simulink model "KUKA_coupled_Dynamics"  (R2023a)
settings: Solver=ode4  StartTime=0.0  StopTime=10  FixedStep=0.01  RelTol=1e-3  EnableMultiTasking=on
InitFcn:
  | % ************** Initiate forces
  | % f0=[0;0;0;0;0;0];
  | % f0=[0;0;0;0;0;0;0];
  | %f_0=[0;0;0];
  | %f_m=[0;0];
  | %f_e=[0;0;0;0;0;0];
  | %iota0=eye(6);
  | % ************** Initiate states
  | %q_m=[2;1];
  | %q_dot_m=[0;1];
  | %P=[0;0;0];
  | %V_I0=[0;0;0];
  | % ************** Load main
  | %run(Main.m)
StopFcn:
  | %format long
  | %table(out.qddot.data(:,1)',out.qddot_ref.data(1,:))
values from neighbouring files (symbols this model uses):
  diag_M = diagonalize(M_frak0, M_frak)    [Create_Robot.m]    (also in Main.m; Main__iiwa7.m; diagonalize.m = zeros(6*(n+1),6*(n+1)); test_C_Main.m)
  f_0 = [0;0;0]    [Create_Robot.m]    (also in Main.m; Main__iiwa7.m = [0;0;0;0;0;0]; test_C_Main.m)
  f_m = [0;0]    [Create_Robot.m]    (also in Main.m; Main__iiwa7.m; test_C_Main.m)
  I0 = eye(3)*416.667    [Create_Robot.m]    (also in Main.m; Main__iiwa7.m = eye(3)*1.66667; test_C_Main.m)
  iota0 = [1 0 0; 0 1 0;zeros(3,3);0 0 1]    [Create_Robot.m]    (also in Main.m = [1 0 0 0 0 0; 0 1 0 0 0 0; 0 0 0 0 0 1]'; Main__iiwa7.m = eye(6,6); test_C_Main.m)
  m0 = 100    [Create_Robot.m]    (also in Main.m; Main__iiwa7.m = 10; test_C_Main.m)
  P = [0;0;0]    [Create_Robot.m]    (also in Main.m = M0*V_I0+M0m*q_dot_m; Main__iiwa7.m = M0*V_I0+M0m*q_dot_m; test_C_Main.m)
  q_dot_m = [0;0]    [Create_Robot.m]    (also in Main.m; Main__iiwa7.m; test_C_Main.m)
  q_m = [0;0]    [Create_Robot.m]    (also in Main.m = [0.2;0.4]; Main__iiwa7.m = [0.2;0.4]; test_C_Main.m = [1;0])
  X = [0 -x(3) x(2) ; x(3) 0 -x(1) ; -x(2) x(1) 0 ]    [skewsym.m]
  Xi_m_matrix = zeros(6*n,n)    [Create_Robot.m]    (also in Main.m; Main__iiwa7.m; test_C_Main.m)
undefined symbols (not defined in the file or in its folder): Xi_m, Y, Z
libraries: sm_lib x80, nesl_utility x36
(part 3 of 3)

== system KUKA_coupled_Dynamics/Space Manipulator1/joint//link6/iiwa_link_6 ==
  Inertia : sm_lib/Body Elements/Inertia  InertiaType=Custom  Mass=2.3466  MassUnits=kg  CenterOfMass=[0, 0, 0]  CenterOfMassUnits=m  MomentsOfInertia=[0.006509, 0.006259, 0.004527]  MomentsOfInertiaUnits=kg*m^2  ProductsOfInertia=[0.00031891, 0, 0]  ProductsOfInertiaUnits=kg*m^2  GraphicType=None  MarkerShape=Inertia  MarkerSize=20  GraphicVisPropType=SimpleVisualProperties  GraphicDiffuseColor=[0.5 0.5 0.5]  GraphicSpecularColor=[0.5 0.5 0.5 1.0]  GraphicAmbientColor=[0.15 0.15 0.15 1.0]  GraphicEmissiveColor=[0.0 0.0 0.0 1.0]  GraphicShininess=75  GraphicOpacity=1.0
  InertiaOriginTransform : sm_lib/Frames and Transforms/Rigid Transform  TranslationMethod=Cartesian  TranslationStandardOffset=0  TranslationStandardOffsetUnits=m  TranslationStandardAxis=+Z  TranslationCartesianOffset=[0, 0.0005999999999999999, 0.0004]  TranslationCartesianOffsetUnits=m  TranslationROffset=0  TranslationROffsetUnits=m  TranslationZOffset=0  TranslationZOffsetUnits=m  TranslationThetaOffset=0  TranslationThetaOffsetUnits=deg  RotationMethod=RotationSequence  RotationAngleUnits=deg  RotationStandardAxis=+Z  RotationAngle=0.0  RotationArbitraryAxis=[0 0 1]  FollAlignAxisA=+X  BaseAlignAxisA=+Y  FollAlignAxisB=+Y  BaseAlignAxisB=+Z  RotationSequenceAxes=BaseAxes  RotationSequence=XYZ  RotationSequenceAngles=[0, 0, 0]  RotationSequenceAnglesUnits=rad  RotationMatrix=[1 0 0; 0 1 0; 0 0 1]  Quaternion=[1 0 0 0]
  ReferenceFrame : sm_lib/Frames and Transforms/Reference Frame
  Visual : sm_lib/Body Elements/File Solid  ExtGeomFileName=iiwa_description/meshes/iiwa7/visual/link_6.stl  UnitType=Custom  ExtGeomFileUnits=m  StepReaderType=HEX  ExportConvexHullGeometry=off  InertiaType=Custom  Mass=0  MassUnits=kg  CenterOfMass=[0, 0, 0]  CenterOfMassUnits=m  MomentsOfInertia=[0, 0, 0]  MomentsOfInertiaUnits=kg*m^2  ProductsOfInertia=[0, 0, 0]  ProductsOfInertiaUnits=kg*m^2  BasedOnType=DensityFromFile  Density=1000  DensityUnits=kg/m^3  DoExposeReferenceFrame=on  SerializedFrames=<Frames/>  GraphicType=FromGeometry  MarkerShape=Sphere  MarkerSize=10  GraphicVisPropType=SimpleVisualProperties  GraphicDiffuseColor=[1, 0.423529411765, 0.0392156862745]  GraphicSpecularColor=[0.5 0.5 0.5 1.0]  GraphicAmbientColor=[0.15 0.15 0.15 1.0]  GraphicEmissiveColor=[0.0 0.0 0.0 1.0]  GraphicShininess=75  GraphicOpacity=1
  VisualOriginTransform : sm_lib/Frames and Transforms/Rigid Transform  TranslationMethod=Cartesian  TranslationStandardOffset=0  TranslationStandardOffsetUnits=m  TranslationStandardAxis=+Z  TranslationCartesianOffset=[0, 0, 0]  TranslationCartesianOffsetUnits=m  TranslationROffset=0  TranslationROffsetUnits=m  TranslationZOffset=0  TranslationZOffsetUnits=m  TranslationThetaOffset=0  TranslationThetaOffsetUnits=deg  RotationMethod=RotationSequence  RotationAngleUnits=deg  RotationStandardAxis=+Z  RotationAngle=0.0  RotationArbitraryAxis=[0 0 1]  FollAlignAxisA=+X  BaseAlignAxisA=+Y  FollAlignAxisB=+Y  BaseAlignAxisB=+Z  RotationSequenceAxes=BaseAxes  RotationSequence=XYZ  RotationSequenceAngles=[0, 0, 0]  RotationSequenceAnglesUnits=rad  RotationMatrix=[1 0 0; 0 1 0; 0 0 1]  Quaternion=[1 0 0 0]
  iiwa_joint_6_AxisInvTransform : sm_lib/Frames and Transforms/Rigid Transform  TranslationMethod=Cartesian  TranslationStandardOffset=0  TranslationStandardOffsetUnits=m  TranslationStandardAxis=+Z  TranslationCartesianOffset=[0, 0, 0]  TranslationCartesianOffsetUnits=m  TranslationROffset=0  TranslationROffsetUnits=m  TranslationZOffset=0  TranslationZOffsetUnits=m  TranslationThetaOffset=0  TranslationThetaOffsetUnits=deg  RotationMethod=ArbitraryAxis  RotationAngleUnits=rad  RotationStandardAxis=+Z  RotationAngle=0  RotationArbitraryAxis=[1, 0, 0]  FollAlignAxisA=+X  BaseAlignAxisA=+Y  FollAlignAxisB=+Y  BaseAlignAxisB=+Z  RotationSequenceAxes=FollowerAxes  RotationSequence=XYX  RotationSequenceAngles=[0 0 0]  RotationSequenceAnglesUnits=deg  RotationMatrix=[1 0 0; 0 1 0; 0 0 1]  Quaternion=[1 0 0 0]
  iiwa_joint_7_AxisTransform : sm_lib/Frames and Transforms/Rigid Transform  TranslationMethod=Cartesian  TranslationStandardOffset=0  TranslationStandardOffsetUnits=m  TranslationStandardAxis=+Z  TranslationCartesianOffset=[0, 0, 0]  TranslationCartesianOffsetUnits=m  TranslationROffset=0  TranslationROffsetUnits=m  TranslationZOffset=0  TranslationZOffsetUnits=m  TranslationThetaOffset=0  TranslationThetaOffsetUnits=deg  RotationMethod=ArbitraryAxis  RotationAngleUnits=rad  RotationStandardAxis=+Z  RotationAngle=0  RotationArbitraryAxis=[1, 0, 0]  FollAlignAxisA=+X  BaseAlignAxisA=+Y  FollAlignAxisB=+Y  BaseAlignAxisB=+Z  RotationSequenceAxes=FollowerAxes  RotationSequence=XYX  RotationSequenceAngles=[0 0 0]  RotationSequenceAnglesUnits=deg  RotationMatrix=[1 0 0; 0 1 0; 0 0 1]  Quaternion=[1 0 0 0]
  iiwa_joint_7_OriginTransform : sm_lib/Frames and Transforms/Rigid Transform  TranslationMethod=Cartesian  TranslationStandardOffset=0  TranslationStandardOffsetUnits=m  TranslationStandardAxis=+Z  TranslationCartesianOffset=[0, 0.081, 0.0607]  TranslationCartesianOffsetUnits=m  TranslationROffset=0  TranslationROffsetUnits=m  TranslationZOffset=0  TranslationZOffsetUnits=m  TranslationThetaOffset=0  TranslationThetaOffsetUnits=deg  RotationMethod=RotationSequence  RotationAngleUnits=deg  RotationStandardAxis=+Z  RotationAngle=0.0  RotationArbitraryAxis=[0 0 1]  FollAlignAxisA=+X  BaseAlignAxisA=+Y  FollAlignAxisB=+Y  BaseAlignAxisB=+Z  RotationSequenceAxes=BaseAxes  RotationSequence=XYZ  RotationSequenceAngles=[-1.57079632679, 3.14159265359, 0]  RotationSequenceAnglesUnits=rad  RotationMatrix=[1 0 0; 0 1 0; 0 0 1]  Quaternion=[1 0 0 0]
  F : PMIOPort  Side=Left
  F1 : PMIOPort  Port=2  Side=Right
  connections:
  Inertia/RConn1 -- InertiaOriginTransform/RConn1
  InertiaOriginTransform/LConn1 -- ReferenceFrame/RConn1 -- VisualOriginTransform/LConn1 -- iiwa_joint_6_AxisInvTransform/LConn1 -- iiwa_joint_7_OriginTransform/LConn1
  Visual/RConn1 -- VisualOriginTransform/RConn1
  iiwa_joint_6_AxisInvTransform/RConn1 -- F/RConn1
  iiwa_joint_7_AxisTransform/RConn1 -- F1/RConn1
  iiwa_joint_7_AxisTransform/LConn1 -- iiwa_joint_7_OriginTransform/RConn1

== system KUKA_coupled_Dynamics/Space Manipulator1/joint//link7/iiwa_link_7 ==
  Inertia : sm_lib/Body Elements/Inertia  InertiaType=Custom  Mass=3.129  MassUnits=kg  CenterOfMass=[0, 0, 0]  CenterOfMassUnits=m  MomentsOfInertia=[0.01464, 0.01465, 0.002872]  MomentsOfInertiaUnits=kg*m^2  ProductsOfInertia=[0, 0, 0.0005912]  ProductsOfInertiaUnits=kg*m^2  GraphicType=None  MarkerShape=Inertia  MarkerSize=20  GraphicVisPropType=SimpleVisualProperties  GraphicDiffuseColor=[0.5 0.5 0.5]  GraphicSpecularColor=[0.5 0.5 0.5 1.0]  GraphicAmbientColor=[0.15 0.15 0.15 1.0]  GraphicEmissiveColor=[0.0 0.0 0.0 1.0]  GraphicShininess=75  GraphicOpacity=1.0
  InertiaOriginTransform : sm_lib/Frames and Transforms/Rigid Transform  TranslationMethod=Cartesian  TranslationStandardOffset=0  TranslationStandardOffsetUnits=m  TranslationStandardAxis=+Z  TranslationCartesianOffset=[0, 0, 0.02]  TranslationCartesianOffsetUnits=m  TranslationROffset=0  TranslationROffsetUnits=m  TranslationZOffset=0  TranslationZOffsetUnits=m  TranslationThetaOffset=0  TranslationThetaOffsetUnits=deg  RotationMethod=RotationSequence  RotationAngleUnits=deg  RotationStandardAxis=+Z  RotationAngle=0.0  RotationArbitraryAxis=[0 0 1]  FollAlignAxisA=+X  BaseAlignAxisA=+Y  FollAlignAxisB=+Y  BaseAlignAxisB=+Z  RotationSequenceAxes=BaseAxes  RotationSequence=XYZ  RotationSequenceAngles=[0, 0, 0]  RotationSequenceAnglesUnits=rad  RotationMatrix=[1 0 0; 0 1 0; 0 0 1]  Quaternion=[1 0 0 0]
  ReferenceFrame : sm_lib/Frames and Transforms/Reference Frame
  Visual : sm_lib/Body Elements/File Solid  ExtGeomFileName=iiwa_description/meshes/iiwa7/visual/link_7.stl  UnitType=Custom  ExtGeomFileUnits=m  StepReaderType=HEX  ExportConvexHullGeometry=off  InertiaType=Custom  Mass=0  MassUnits=kg  CenterOfMass=[0, 0, 0]  CenterOfMassUnits=m  MomentsOfInertia=[0, 0, 0]  MomentsOfInertiaUnits=kg*m^2  ProductsOfInertia=[0, 0, 0]  ProductsOfInertiaUnits=kg*m^2  BasedOnType=DensityFromFile  Density=1000  DensityUnits=kg/m^3  DoExposeReferenceFrame=on  SerializedFrames=<Frames/>  GraphicType=FromGeometry  MarkerShape=Sphere  MarkerSize=10  GraphicVisPropType=SimpleVisualProperties  GraphicDiffuseColor=[0.4, 0.4, 0.4]  GraphicSpecularColor=[0.5 0.5 0.5 1.0]  GraphicAmbientColor=[0.15 0.15 0.15 1.0]  GraphicEmissiveColor=[0.0 0.0 0.0 1.0]  GraphicShininess=75  GraphicOpacity=1
  VisualOriginTransform : sm_lib/Frames and Transforms/Rigid Transform  TranslationMethod=Cartesian  TranslationStandardOffset=0  TranslationStandardOffsetUnits=m  TranslationStandardAxis=+Z  TranslationCartesianOffset=[0, 0, -0.0005]  TranslationCartesianOffsetUnits=m  TranslationROffset=0  TranslationROffsetUnits=m  TranslationZOffset=0  TranslationZOffsetUnits=m  TranslationThetaOffset=0  TranslationThetaOffsetUnits=deg  RotationMethod=RotationSequence  RotationAngleUnits=deg  RotationStandardAxis=+Z  RotationAngle=0.0  RotationArbitraryAxis=[0 0 1]  FollAlignAxisA=+X  BaseAlignAxisA=+Y  FollAlignAxisB=+Y  BaseAlignAxisB=+Z  RotationSequenceAxes=BaseAxes  RotationSequence=XYZ  RotationSequenceAngles=[0, 0, 0]  RotationSequenceAnglesUnits=rad  RotationMatrix=[1 0 0; 0 1 0; 0 0 1]  Quaternion=[1 0 0 0]
  iiwa_joint_7_AxisInvTransform : sm_lib/Frames and Transforms/Rigid Transform  TranslationMethod=Cartesian  TranslationStandardOffset=0  TranslationStandardOffsetUnits=m  TranslationStandardAxis=+Z  TranslationCartesianOffset=[0, 0, 0]  TranslationCartesianOffsetUnits=m  TranslationROffset=0  TranslationROffsetUnits=m  TranslationZOffset=0  TranslationZOffsetUnits=m  TranslationThetaOffset=0  TranslationThetaOffsetUnits=deg  RotationMethod=ArbitraryAxis  RotationAngleUnits=rad  RotationStandardAxis=+Z  RotationAngle=0  RotationArbitraryAxis=[1, 0, 0]  FollAlignAxisA=+X  BaseAlignAxisA=+Y  FollAlignAxisB=+Y  BaseAlignAxisB=+Z  RotationSequenceAxes=FollowerAxes  RotationSequence=XYX  RotationSequenceAngles=[0 0 0]  RotationSequenceAnglesUnits=deg  RotationMatrix=[1 0 0; 0 1 0; 0 0 1]  Quaternion=[1 0 0 0]
  iiwa_joint_ee_OriginTransform : sm_lib/Frames and Transforms/Rigid Transform  TranslationMethod=Cartesian  TranslationStandardOffset=0  TranslationStandardOffsetUnits=m  TranslationStandardAxis=+Z  TranslationCartesianOffset=[0, 0, 0.045]  TranslationCartesianOffsetUnits=m  TranslationROffset=0  TranslationROffsetUnits=m  TranslationZOffset=0  TranslationZOffsetUnits=m  TranslationThetaOffset=0  TranslationThetaOffsetUnits=deg  RotationMethod=RotationSequence  RotationAngleUnits=deg  RotationStandardAxis=+Z  RotationAngle=0.0  RotationArbitraryAxis=[0 0 1]  FollAlignAxisA=+X  BaseAlignAxisA=+Y  FollAlignAxisB=+Y  BaseAlignAxisB=+Z  RotationSequenceAxes=BaseAxes  RotationSequence=XYZ  RotationSequenceAngles=[0, -1.57079632679, 0]  RotationSequenceAnglesUnits=rad  RotationMatrix=[1 0 0; 0 1 0; 0 0 1]  Quaternion=[1 0 0 0]
  iiwa_joint_ee_kuka_OriginTransform : sm_lib/Frames and Transforms/Rigid Transform  TranslationMethod=Cartesian  TranslationStandardOffset=0  TranslationStandardOffsetUnits=m  TranslationStandardAxis=+Z  TranslationCartesianOffset=[0, 0, 0.045]  TranslationCartesianOffsetUnits=m  TranslationROffset=0  TranslationROffsetUnits=m  TranslationZOffset=0  TranslationZOffsetUnits=m  TranslationThetaOffset=0  TranslationThetaOffsetUnits=deg  RotationMethod=RotationSequence  RotationAngleUnits=deg  RotationStandardAxis=+Z  RotationAngle=0.0  RotationArbitraryAxis=[0 0 1]  FollAlignAxisA=+X  BaseAlignAxisA=+Y  FollAlignAxisB=+Y  BaseAlignAxisB=+Z  RotationSequenceAxes=BaseAxes  RotationSequence=XYZ  RotationSequenceAngles=[3.14159265359, 3.14159265359, 3.14159265359]  RotationSequenceAnglesUnits=rad  RotationMatrix=[1 0 0; 0 1 0; 0 0 1]  Quaternion=[1 0 0 0]
  F : PMIOPort  Side=Left
  F2 : PMIOPort  Port=2  Side=Right
  F1 : PMIOPort  Port=3  Side=Right
  connections:
  Inertia/RConn1 -- InertiaOriginTransform/RConn1
  InertiaOriginTransform/LConn1 -- iiwa_joint_ee_OriginTransform/LConn1 -- iiwa_joint_ee_kuka_OriginTransform/LConn1 -- iiwa_joint_7_AxisInvTransform/LConn1 -- VisualOriginTransform/LConn1 -- ReferenceFrame/RConn1
  Visual/RConn1 -- VisualOriginTransform/RConn1
  iiwa_joint_7_AxisInvTransform/RConn1 -- F/RConn1
  iiwa_joint_ee_OriginTransform/RConn1 -- F1/RConn1
  iiwa_joint_ee_kuka_OriginTransform/RConn1 -- F2/RConn1

== system KUKA_coupled_Dynamics/old model1/Inverse Dynamics/Euler Poincare ==
  P : Inport
  V : Inport  Port=2
  f_0 : Inport  Port=3
  Add : Sum  Inputs=+-
  Constant : Constant  Value=iota0
  MATLAB Function : MATLAB Function  TreatAsAtomicUnit=on
  Matrix Multiply : Product  Multiplication=Matrix(*)
  To Workspace : ToWorkspace  VariableName=simout  SaveFormat=Timeseries  SampleTime=-1
  Transpose : Math  Operator=transpose
  P_dot : Outport
  wires:
  P/1 -> Matrix Multiply/2
  MATLAB Function/1(adj_low) -> Transpose/1
  V/1 -> MATLAB Function/1(V)
  Transpose/1 -> To Workspace/1, Matrix Multiply/1
  Matrix Multiply/1 -> Add/1
  f_0/1 -> Add/2
  Add/1 -> P_dot/1
  Constant/1 -> MATLAB Function/2(iota0)

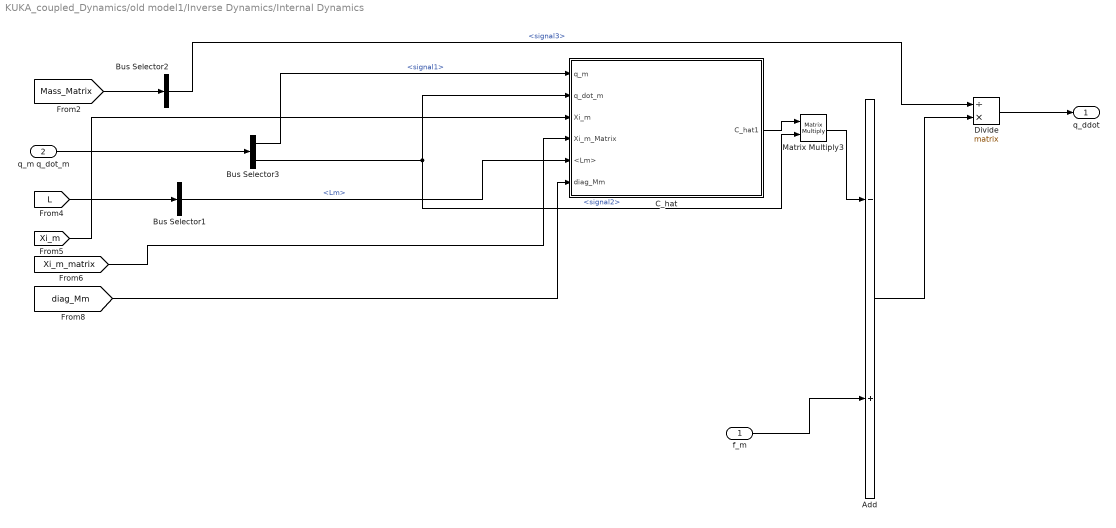
== system KUKA_coupled_Dynamics/old model1/Inverse Dynamics/Internal Dynamics ==
  f_m : Inport
  q_m q_dot_m : Inport  Port=2
  Add : Sum  Inputs=-+
  Bus Selector1 : BusSelector  OutputSignals=Lm
  Bus Selector2 : BusSelector  OutputSignals=signal3
  Bus Selector3 : BusSelector  OutputSignals=signal1,signal2
  C_hat : Subsystem
  Divide : Product  Inputs=/*  Multiplication=Matrix(*)
  Matrix Multiply3 : Product  Multiplication=Matrix(*)
  q_ddot : Outport
  wires:
  f_m/1 -> Add/2
  Divide/1 -> q_ddot/1
  q_m q_dot_m/1 -> Bus Selector3/1
  [Mass_Matrix] -> Bus Selector2/1
  [L] -> Bus Selector1/1
  [Xi_m] -> C_hat/3(Xi_m)
  [Xi_m_matrix] -> C_hat/4(Xi_m_Matrix)
  [diag_Mm] -> C_hat/6(diag_Mm)
  C_hat/1(C_hat1) -> Matrix Multiply3/1
  Matrix Multiply3/1 -> Add/1
  Add/1 -> Divide/2
  Bus Selector3/2 -> Matrix Multiply3/2, C_hat/2(q_dot_m)  "<signal2>"
  Bus Selector3/1 -> C_hat/1(q_m)  "<signal1>"
  Bus Selector1/1 -> C_hat/5(<Lm>)  "<Lm>"
  Bus Selector2/1 -> Divide/1  "<signal3>"

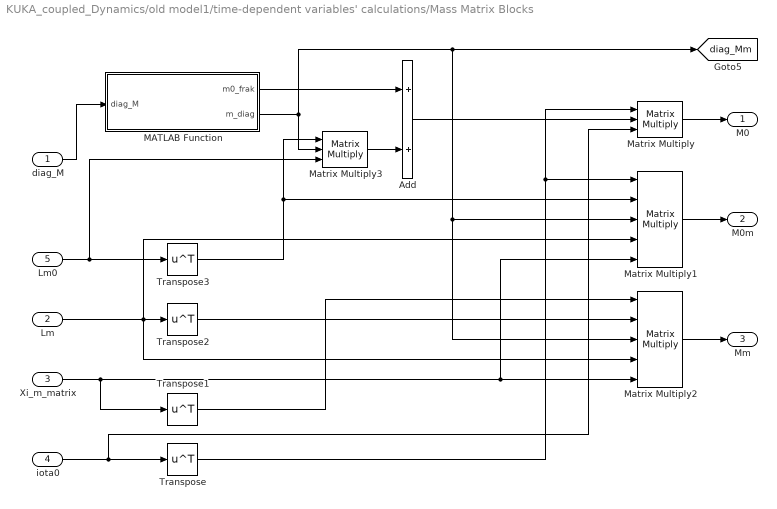
== system KUKA_coupled_Dynamics/old model1/time-dependent variables' calculations/Mass Matrix Blocks ==
  diag_M : Inport
  Lm : Inport  Port=2
  Xi_m_matrix : Inport  Port=3
  iota0 : Inport  Port=4
  Lm0 : Inport  Port=5
  Add : Sum
  MATLAB Function : MATLAB Function  TreatAsAtomicUnit=on
  Matrix Multiply : Product  Inputs=3  Multiplication=Matrix(*)
  Matrix Multiply1 : Product  Inputs=5  Multiplication=Matrix(*)
  Matrix Multiply2 : Product  Inputs=5  Multiplication=Matrix(*)
  Matrix Multiply3 : Product  Inputs=3  Multiplication=Matrix(*)
  Transpose{,1..3} (4 alike) : Math  Operator=transpose
  M0 : Outport
  M0m : Outport  Port=2
  Mm : Outport  Port=3
  tag scope: diag_Mm=global
  wires:
  Matrix Multiply2/1 -> Mm/1
  Xi_m_matrix/1 -> Transpose1/1, Matrix Multiply1/5, Matrix Multiply2/5
  diag_M/1 -> MATLAB Function/1(diag_M)
  Lm/1 -> Matrix Multiply2/4, Matrix Multiply1/4, Transpose2/1
  Transpose1/1 -> Matrix Multiply2/1
  Transpose2/1 -> Matrix Multiply2/2
  MATLAB Function/2(m_diag) -> Matrix Multiply1/3, Matrix Multiply2/3, [diag_Mm], Matrix Multiply3/2
  Matrix Multiply1/1 -> M0m/1
  Matrix Multiply/1 -> M0/1
  iota0/1 -> Matrix Multiply/3, Transpose/1
  Transpose/1 -> Matrix Multiply/1, Matrix Multiply1/1
  Add/1 -> Matrix Multiply/2
  Matrix Multiply3/1 -> Add/2
  MATLAB Function/1(m0_frak) -> Add/1
  Lm0/1 -> Matrix Multiply3/3, Transpose3/1
  Transpose3/1 -> Matrix Multiply1/2, Matrix Multiply3/1

== system KUKA_coupled_Dynamics/Inverse Dynamics2/Internal Dynamics/C_hat/Lm_partials ==
  q_m : Inport
  Xi_m : Inport  Port=2
  Constant : Constant  Value=iota0
  Lm0partial : MATLAB Function  TreatAsAtomicUnit=on
  Lmpartial : MATLAB Function  TreatAsAtomicUnit=on
  Lm_partial : Outport
  Lm0_partial : Outport  Port=2
  wires:
  Lmpartial/1(Lm_partial) -> Lm_partial/1
  Lm0partial/1(Lm0_partial) -> Lm0_partial/1
  Constant/1 -> Lm0partial/3(iota0), Lmpartial/3(iota0)
  q_m/1 -> Lm0partial/1(q_m), Lmpartial/1(q_m)
  Xi_m/1 -> Lm0partial/2(Xi_m), Lmpartial/2(Xi_m)

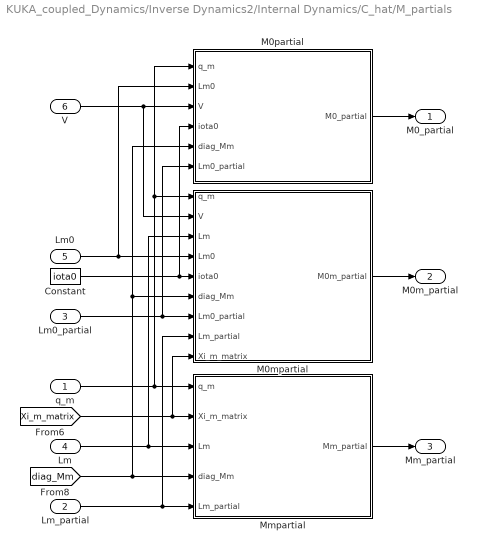
== system KUKA_coupled_Dynamics/Inverse Dynamics2/Internal Dynamics/C_hat/M_partials ==
  q_m : Inport
  Lm_partial : Inport  Port=2
  Lm0_partial : Inport  Port=3
  Lm : Inport  Port=4
  Lm0 : Inport  Port=5
  V : Inport  Port=6
  " M0partial" : MATLAB Function  TreatAsAtomicUnit=on
  Constant : Constant  Value=iota0
  M0mpartial : MATLAB Function  TreatAsAtomicUnit=on
  Mmpartial : MATLAB Function  TreatAsAtomicUnit=on
  M0_partial : Outport
  M0m_partial : Outport  Port=2
  Mm_partial : Outport  Port=3
  wires:
  Lm_partial/1 -> M0mpartial/8(Lm_partial), Mmpartial/5(Lm_partial)
  q_m/1 -> " M0partial"/1(q_m), M0mpartial/1(q_m), Mmpartial/1(q_m)
  [diag_Mm] -> " M0partial"/5(diag_Mm), M0mpartial/6(diag_Mm), Mmpartial/4(diag_Mm)
  [Xi_m_matrix] -> M0mpartial/9(Xi_m_matrix), Mmpartial/2(Xi_m_matrix)
  Lm/1 -> M0mpartial/3(Lm), Mmpartial/3(Lm)
  Mmpartial/1(Mm_partial) -> Mm_partial/1
  M0mpartial/1(M0m_partial) -> M0m_partial/1
  " M0partial"/1(M0_partial) -> M0_partial/1
  Lm0/1 -> " M0partial"/2(Lm0), M0mpartial/4(Lm0)
  Lm0_partial/1 -> " M0partial"/6(Lm0_partial), M0mpartial/7(Lm0_partial)
  Constant/1 -> " M0partial"/4(iota0), M0mpartial/5(iota0)
  V/1 -> M0mpartial/2(V), " M0partial"/3(V)

== system KUKA_coupled_Dynamics/old model1/Inverse Dynamics/Internal Dynamics/C_hat ==
  q_m : Inport
  q_dot_m : Inport  Port=2
  Xi_m : Inport  Port=3
  Xi_m_Matrix : Inport  Port=4
  <Lm> : Inport  Port=5
  diag_Mm : Inport  Port=6
  C_hat : MATLAB Function  TreatAsAtomicUnit=on
  Lm_partials : Subsystem
  M_partials : Subsystem
  C_hat1 : Outport
  wires:
  C_hat/1(C_hat) -> C_hat1/1
  q_m/1 -> C_hat/1(q_m), M_partials/1(q_m), Lm_partials/1(q_m)
  q_dot_m/1 -> C_hat/2(q_dot_m)
  Xi_m_Matrix/1 -> M_partials/3(Xi_m_Matrix)
  <Lm>/1 -> M_partials/4(Lm)
  diag_Mm/1 -> M_partials/5(diag_Mm)
  Xi_m/1 -> Lm_partials/2(Xi_m)
  Lm_partials/1(Lm_partial) -> M_partials/2(Lm_partial)
  M_partials/1(Mm_partial) -> C_hat/3(Mm_hat_partial)

== system KUKA_coupled_Dynamics/old model1/Inverse Dynamics/Internal Dynamics/C_hat/Lm_partials ==
  q_m : Inport
  Xi_m : Inport  Port=2
  Constant : Constant  Value=iota0
  Lmpartial : MATLAB Function  TreatAsAtomicUnit=on
  Lm_partial : Outport
  wires:
  Xi_m/1 -> Lmpartial/2(Xi_m)
  q_m/1 -> Lmpartial/1(q_m)
  Lmpartial/1(Lm_partial) -> Lm_partial/1
  Constant/1 -> Lmpartial/3(iota0)

== system KUKA_coupled_Dynamics/old model1/Inverse Dynamics/Internal Dynamics/C_hat/M_partials ==
  q_m : Inport
  Lm_partial : Inport  Port=2
  Xi_m_Matrix : Inport  Port=3
  Lm : Inport  Port=4
  diag_Mm : Inport  Port=5
  Mmpartial : MATLAB Function  TreatAsAtomicUnit=on
  Mm_partial : Outport
  wires:
  Lm_partial/1 -> Mmpartial/5(Lm_partial)
  q_m/1 -> Mmpartial/1(q_m)
  diag_Mm/1 -> Mmpartial/4(diag_Mm)
  Xi_m_Matrix/1 -> Mmpartial/2(Xi_m_Matrix)
  Lm/1 -> Mmpartial/3(Lm)
  Mmpartial/1(Mm_partial) -> Mm_partial/1

== matlab function KUKA_coupled_Dynamics/Inverse Dynamics2/Internal Dynamics/C_hat/M_partials/M0mpartial ==
  data: q_m input; M0m_partial output; V input; Lm input; Lm0 input; iota0 input; diag_Mm input; Lm0_partial input; Lm_partial input; Xi_m_matrix input
function M0m_partial = M0m_partial(q_m,V,Lm,Lm0,iota0,diag_Mm,Lm0_partial,Lm_partial, Xi_m_matrix)
% Calculates the C_hat_m matrix from base pose and arm joint angles

n=length(q_m);
b=length(V);

% Find partial of M0m to joint angles
M0m_partial=zeros(b,n,n);
for i=1:n
    temp1=transpose(Lm0_partial(1:end,1:end,i))*diag_Mm*Lm;
    temp2=transpose(Lm0)*diag_Mm*Lm_partial(1:end,1:end,i);
    M0m_partial(1:b,1:n,i)= iota0'*(temp1+temp2)*Xi_m_matrix; % equation 118 of TRO paper
end

== matlab function KUKA_coupled_Dynamics/Inverse Dynamics2/Internal Dynamics/C_hat/M_partials/Mmpartial ==
  data: q_m input; Mm_partial output; Xi_m_matrix input; Lm input; diag_Mm input; Lm_partial input
function Mm_partial = Mm_partial(q_m,Xi_m_matrix,Lm,diag_Mm,Lm_partial)
% Calculates the C_hat_m matrix from base pose and arm joint angles

n=length(q_m);

% find the non-generalized arm mass matrix'x derivative to joint angles
Mm_partial=zeros(n,n,n);
for i=1:n
    temp=   transpose(Lm_partial(1:6*n,1:6*n,i))*diag_Mm*Lm  +   transpose(Lm)*diag_Mm*Lm_partial(1:6*n,1:6*n,i);
    Mm_partial(1:n,1:n,i)=transpose(Xi_m_matrix)*temp*Xi_m_matrix; %calcualte the derivative of not-augmented arm mass matrix from equation 120 of TRO paper
end

== matlab function KUKA_coupled_Dynamics/Inverse Dynamics2/Internal Dynamics/C_hat/Mm_hat_partial ==
  data: q_m input; AMA_partial input; Mm_hat_partial output; Mm_partial input
function Mm_hat_partial = Mm_hat_partial(q_m, AMA_partial, Mm_partial)
% Calculates the C_hat_m matrix from base pose and arm joint angles

n=length(q_m);

% find the generalized arm mass matrix'x derivative to joint angles
Mm_hat_partial=zeros(n,n,n);
for i=1:n
    Mm_hat_partial(1:n,1:n,i)=Mm_partial(1:n,1:n,i)-AMA_partial(1:n,1:n,i); %calcualte the derivative of augmented arm mass matrix from equation 119 of TRO paper
end

== matlab function KUKA_coupled_Dynamics/Inverse Dynamics2/Internal Dynamics/M_hat ==
  data: M0 input; Mm input; A input; M_hat output
function M_hat =M_hat(M0,Mm,A)
% Compute the Mass Matrix of the multibody system.
%   Input:
%   M0      Spacecraft mass matrix 
%   M0m     Coupling
%   Mm      Manipulator mass matrix

% Calculate M_hat
M_hat=Mm-transpose(A)*M0*A;


end

== matlab function KUKA_coupled_Dynamics/old model1/Inverse Dynamics/Euler Poincare/MATLAB Function ==
  data: V input; adj_low output; iota0 input
function adj_low = adj_low(V, iota0)
% calculates the adjoint corresponding to the Lie bracket of vector V and ()
adj_low = adjoint_low(V,iota0);

== matlab function KUKA_coupled_Dynamics/old model1/Inverse Dynamics/Internal Dynamics/C_hat/C_hat ==
  data: q_m input; q_dot_m input; C_hat output; Mm_hat_partial input
function C_hat = C_hat(q_m,q_dot_m, Mm_hat_partial)
% Calculates the C_hat_m matrix from base pose and arm joint angles

n=length(q_m);


% Calculate C_hat matrix
C_temp1=zeros(n,n);
C_temp2=zeros(n,n);
C_hat=zeros(n,n);
for i=1:n
    C_temp1=C_temp1+Mm_hat_partial(1:n,1:n,i).*q_dot_m(i); % nxn by scalar
    C_temp2(i,1:n)=0.5*transpose(q_dot_m)*Mm_hat_partial(1:n,1:n,i); %1xn by nxn 
end

C_hat=C_temp1-C_temp2;

== matlab function KUKA_coupled_Dynamics/old model1/Inverse Dynamics/Internal Dynamics/C_hat/Lm_partials/Lmpartial ==
  data: q_m input; Lm_partial output; Xi_m input; iota0 input
function Lm_partial  = Lm_partial(q_m,Xi_m,iota0)
% Calculates the C_hat_m matrix from base pose and arm joint angles

n=length(q_m);

% Find partial of Lm0 to joint angles
Lm_partial=zeros(6*n,6*n,n); % 6nx6xn
for i=1:n
    for j=1:n
        for k=1:n
            if j==k
                Lm_partial(6*(j-1)+1:6*(j-1)+6,6*(k-1)+1:6*(k-1)+6,i)=eye(6,6);
            elseif j>i && i>=k
                Lm_partial(6*(j-1)+1:6*j,6*(k-1)+1:6*k,i)=-Ad_frak(j,i+1,Xi_m,q_m)*adjoint_low(Xi_m(:,i),iota0)*Ad_frak(i,k,Xi_m,q_m); % equation 81 of TRO paper
            elseif i==j && i>=k
                Lm_partial(6*(j-1)+1:6*j,6*(k-1)+1:6*k,i)=-adjoint_low(Xi_m(:,i),iota0)*Ad_frak(i,k,Xi_m,q_m); % equation 81 of TRO paper
            else
                Lm_partial(6*(j-1)+1:6*(j-1)+6,6*(k-1)+1:6*(k-1)+6,i)=zeros(6,6);
            end

        end
    end
end

== matlab function KUKA_coupled_Dynamics/old model1/Inverse Dynamics/Internal Dynamics/C_hat/M_partials/Mmpartial ==
  data: q_m input; Mm_partial output; Xi_m_Matrix input; Lm input; diag_Mm input; Lm_partial input
function Mm_partial = Mm_partial(q_m,Xi_m_Matrix,Lm,diag_Mm,Lm_partial)
% Calculates the C_hat_m matrix from base pose and arm joint angles

n=length(q_m);

% find the non-generalized arm mass matrix'x derivative to joint angles
Mm_partial=zeros(n,n,n);
for i=1:n
    Mm_partial(1:n,1:n,i)=transpose(Xi_m_Matrix)*(transpose(Lm_partial(1:6*n,1:6*n,i))*diag_Mm*Lm + ...
        transpose(Lm)*diag_Mm*Lm_partial(1:6*n,1:6*n,i))*Xi_m_Matrix; %calcualte the derivative of not-augmented arm mass matrix from equation 120 of TRO paper
end

== matlab function KUKA_coupled_Dynamics/old model1/time-dependent variables' calculations/  ==
  data: q_m input; L0 output; Lm0 output; Lm output; Xi_m input
function [L0,Lm0,Lm] =L_calculator(q_m,Xi_m)
% Calculates the time-dependent L matrix
n=length(q_m);
L=zeros(6*(n+1),6*(n+1));
% Compute M_frak for ith body
% Calculate L matrix
for i=1:n+1
    for j=1:n+1
        if i>j
            Ad_temp=eye(6);
            for k=j:i-1
                Ad_temp=Adjoint(g_Matrix(-Xi_m(:,k),q_m(k)))*Ad_temp;
            end
            L(6*(i-1)+1:6*(i-1)+6,6*(j-1)+1:6*(j-1)+6)=Ad_temp;
        elseif i==j
            L(6*(i-1)+1:6*(i-1)+6,6*(j-1)+1:6*(j-1)+6)=eye(6);
        elseif i<j
            L(6*(i-1)+1:6*(i-1)+6,6*(j-1)+1:6*(j-1)+6)=zeros(6);
        end
    end
end

L0=L(1:6,1:6);
Lm0=L(7:end,1:6);
Lm=L(7:end,7:end);

end

== matlab function KUKA_coupled_Dynamics/old model1/time-dependent variables' calculations/MATLAB Function ==
  data: M0 input; M0m input; A output
function A=A_connection(M0,M0m)
% Compute the connection A from mass properties

A=M0\M0m;

== matlab function KUKA_coupled_Dynamics/old model1/time-dependent variables' calculations/Mass Matrix Blocks/MATLAB Function ==
  data: diag_M input; m0_frak output; m_diag output
function [m0_frak,m_diag]=m_frak_decomp(diag_M)
% Compute the Mass Matrix of the multibody system.
%   Output:
%   M0      Spacecraft mass matrix 
%   M0m
%   Mm      Manipulator mass matrix

%n=length(q_m);

m0_frak=diag_M(1:6,1:6);
m_diag=diag_M(7:end,7:end);

== matlab function KUKA_coupled_Dynamics/old model1/time-dependent variables' calculations/V_I0 ==
  data: P input; A_connection input; q_dot_m input; M0 input; V_I0 output
function V_I0=V_I0(P,A_connection,q_dot_m,M0)
% Find the spaccecraft velocity V_I0
% M0_inv=inv(M0);
% temp=P-transpose(A_connection)*q_dot_m;
V_I0=M0\P-A_connection*q_dot_m;

== matlab function KUKA_coupled_Dynamics/time-dependent variables' calculations2/  ==
  data: q_m input; L0 output; Lm0 output; Lm output; Xi_m input
function [L0,Lm0,Lm] =L_calculator(q_m,Xi_m)
% Calculates the time-dependent L matrix
n=length(q_m);
L=zeros(6*(n+1),6*(n+1));
% Compute M_frak for ith body
% Calculate L matrix
for i=1:n+1
    for j=1:n+1
        if i>j
            Ad_temp=eye(6);
            for k=j:i-1
                Ad_temp=Adjoint(g_Matrix(-Xi_m(:,k),q_m(k)))*Ad_temp;
            end
            L(6*(i-1)+1:6*(i-1)+6,6*(j-1)+1:6*(j-1)+6)=Ad_temp;
        elseif i==j
            L(6*(i-1)+1:6*(i-1)+6,6*(j-1)+1:6*(j-1)+6)=eye(6);
        elseif i<j
            L(6*(i-1)+1:6*(i-1)+6,6*(j-1)+1:6*(j-1)+6)=zeros(6);
        end
    end
end

L0=L(1:6,1:6);
Lm0=L(7:end,1:6);
Lm=L(7:end,7:end);

end

== matlab function KUKA_coupled_Dynamics/time-dependent variables' calculations2/MATLAB Function ==
  data: M0 input; M0m input; A output
function A=A_connection(M0,M0m)
% Compute the connection A from mass properties

A=M0\M0m;

== matlab function KUKA_coupled_Dynamics/time-dependent variables' calculations2/Mass Matrix Blocks/MATLAB Function ==
  data: diag_M input; m0_frak output; m_diag output
function [m0_frak,m_diag]=m_frak_decomp(diag_M)
% Compute the Mass Matrix of the multibody system.
%   Output:
%   M0      Spacecraft mass matrix 
%   M0m
%   Mm      Manipulator mass matrix

%n=length(q_m);

m0_frak=diag_M(1:6,1:6);
m_diag=diag_M(7:end,7:end);

== matlab function KUKA_coupled_Dynamics/time-dependent variables' calculations2/V_I0 ==
  data: P input; A_connection input; q_dot_m input; M0 input; V_I0 output
function V_I0=V_I0(P,A_connection,q_dot_m,M0)
% Find the spaccecraft velocity V_I0
% M0_inv=inv(M0);
% temp=P-transpose(A_connection)*q_dot_m;
V_I0=M0\P-A_connection*q_dot_m;

== matlab function KUKA_coupled_Dynamics/time-dependent variables' calculations2/degree zeroer ==
  data: q_m input; q output
function q=degreezeroer(q_m)
q=q_m;
n=length(q(:,1));
for i=1:n
    if q(i)>0
        while q(i)>2*pi
            q(i)=q(i)-2*pi;
        end
    elseif q(i)<0
        while q(i)<-2*pi
            q(i)=q(i)+2*pi;
        end
    end
end
end

== matlab function KUKA_coupled_Dynamics/Inverse Dynamics2/Internal Dynamics/N_hat/N_hat ==
  data: N_hat_temp output; q_m input; q_dot_m input; A input; V input; P input; M0_partial input; A_partial input; iota0 input; M0 input
function N_hat_temp = N_hat(q_m,q_dot_m,A,V,P,M0_partial, A_partial, iota0, M0)
% Calculates the N_hat_m matrix from base pose and arm joint angles

n=length(q_m);
b=length(V);

%Form N_hat from equation 19 of ACC paper
N_temp1=zeros(n,b); N_temp2=zeros(n,b); N_temp3=zeros(n,b);

for i=1:n
    N_temp1=N_temp1+transpose(squeeze(A_partial(1:b,1:n,i)).*q_dot_m(i)); % transpose of (bxn times 1x1) 
    N_temp2(i,1:b)=transpose(q_dot_m)*transpose(squeeze(A_partial(1:b,1:n,i))); %1xn times nxb
    N_temp3(i,1:b)=0.5*transpose(P)*(-M0\M0_partial(1:end,1:end,i)/M0); % 1xb times bxb
end

N_hat_temp=transpose(A)*transpose(adjoint_low(V,iota0))-N_temp1+N_temp2+N_temp3;

== matlab function KUKA_coupled_Dynamics/Inverse Dynamics2/Euler Poincare/adj_low_P ==
  data: P input; adj_low output; iota0 input
function adj_low = adj_low(P, iota0)
% calculates the adjoint corresponding to the Lie bracket of vector V and ()
adj_low = adjoint_low_momentum(P,iota0);

== matlab function KUKA_coupled_Dynamics/Inverse Dynamics2/Euler Poincare/MATLAB Function ==
  data: V input; adj_low output; iota0 input
function adj_low = adj_low(V, iota0)
% calculates the adjoint corresponding to the Lie bracket of vector V and ()
adj_low = adjoint_low(V,iota0);

== matlab function KUKA_coupled_Dynamics/Inverse Dynamics2/Internal Dynamics/C_hat/AMA_partial ==
  data: q_m input; AMA_partial output; M0 input; A input; A_partial input; V input; M0_partial input
function AMA_partial = AMA_partial(q_m,M0,A,A_partial,V,M0_partial)
% Calculates the C_hat_m matrix from base pose and arm joint angles

n=length(q_m);
b=length(V);

% find the temp intermediate term
AMA_partial=zeros(n,n,n);
for i=1:n
    AMA_partial(1:n,1:n,i)=transpose(A_partial(1:end,1:end,i))*M0*A+transpose(A)*M0_partial(1:end,1:end,i)*A+transpose(A)*M0*A_partial(1:end,1:end,i); %calcualte the derivative of not-augmented arm mass matrix from equation 121 of TRO paper
end

== matlab function KUKA_coupled_Dynamics/Inverse Dynamics2/Internal Dynamics/C_hat/A_partial ==
  data: q_m input; A_partial output; M0 input; M0_partial input; M0m_partial input; M0m input; V input
function A_partial = A_partial(q_m,M0,M0_partial,M0m_partial,M0m,V)
% Calculates the C_hat_m matrix from base pose and arm joint angles

n=length(q_m);
b=length(V);

% Find partial of connection A to each joint angle
A_partial=zeros(b,n,n);

temp1=zeros(b,n);
temp2=zeros(b,n);
temp3=zeros(b,n);

for i=1:n
    temp1=M0\M0_partial(1:end,1:end,i);
    temp2=M0\M0m;
    temp3=M0\M0m_partial(1:end,1:end,i);
    A_partial(1:b,1:n,i)=-temp1*temp2+temp3; % Equation 122
end

== matlab function KUKA_coupled_Dynamics/Inverse Dynamics2/Internal Dynamics/C_hat/C_hat ==
  data: q_m input; Mm_hat_partial input; q_dot_m input; C_hat output
function C_hat = C_hat(q_m, Mm_hat_partial,q_dot_m)
% Calculates the C_hat_m matrix from base pose and arm joint angles

n=length(q_m);


% Calculate C_hat matrix
C_temp1=zeros(n,n);
C_temp2=zeros(n,n);
C_hat=zeros(n,n);
for i=1:n
    C_temp1=C_temp1+squeeze(Mm_hat_partial(1:n,1:n,i)).*q_dot_m(i); % nxn by scalar
    C_temp2(i,1:n)=0.5*transpose(q_dot_m)*squeeze(Mm_hat_partial(1:n,1:n,i)); %1xn by nxn 
end

C_hat=C_temp1-C_temp2;

== matlab function KUKA_coupled_Dynamics/Inverse Dynamics2/Internal Dynamics/C_hat/Lm_partials/Lm0partial ==
  data: q_m input; Lm0_partial output; Xi_m input; iota0 input
function Lm0_partial = Lm0_partial(q_m,Xi_m,iota0)
% Calculates the C_hat_m matrix from base pose and arm joint angles

n=length(q_m);

% Find partial of Lm to joint angles
Lm0_partial=zeros(6*n,6,n); % 6nx6xn
for i=1:n
    for j=1:n
        Lm0_partial(6*(j-1)+1:6*j,1:6,i)=Ad_partial(j,1,i,Xi_m,q_m,iota0); % equation 114 of TRO paper
    end
end

%%%%%%%%%%%%%%%%%%%%%%%%%%%%%%%%%%%%%%%%%%%%%%%%%%%%%%%%%%%%% MUST BE
%%%%%%%%%%%%%%%%%%%%%%%%%%%%%%%%%%%%%%%%%%%%%%%%%%%%%%%%%%%%% CHECKED

== matlab function KUKA_coupled_Dynamics/Inverse Dynamics2/Internal Dynamics/C_hat/Lm_partials/Lmpartial ==
  data: q_m input; Lm_partial output; Xi_m input; iota0 input
function Lm_partial  = Lm_partial(q_m,Xi_m,iota0)
% Calculates the C_hat_m matrix from base pose and arm joint angles

n=length(q_m);

% Find partial of Lm0 to joint angles
Lm_partial=zeros(6*n,6*n,n); % 6nx6xn
for i=1:n
    Lm_partial(:,:,i)=zeros(6*n,6*n);
    for j=2:n
        for k=2:n
            if j>i && i>=k
                Lm_partial(6*(j-1)+1:6*j,6*(k-2)+1:6*(k-1),i)=Ad_partial(j,k,i,Xi_m,q_m,iota0); % equation 81 of TRO paper
            elseif i==j && i>=k
                Lm_partial(6*(j-1)+1:6*j,6*(k-2)+1:6*(k-1),i)=Ad_partial(j,k,i,Xi_m,q_m,iota0); % equation 81 of TRO paper
            else
                Lm_partial(6*(j-1)+1:6*(j-1)+6,6*(k-2)+1:6*(k-2)+6,i)=zeros(6,6);
            end

        end
    end
end

== matlab function KUKA_coupled_Dynamics/Inverse Dynamics2/Internal Dynamics/C_hat/M_partials/ M0partial ==
  data: q_m input; M0_partial output; Lm0 input; V input; iota0 input; diag_Mm input; Lm0_partial input
function M0_partial = M0_partial(q_m,Lm0,V,iota0,diag_Mm,Lm0_partial)
% Calculates the C_hat_m matrix from base pose and arm joint angles

n=length(q_m);
b=length(V);

% Find partial of M0 to joint angles
M0_partial=zeros(b,b,n); %initiate
for i=1:n
    temp1=transpose(Lm0_partial(1:end,1:end,i))*diag_Mm*Lm0;
    temp2=transpose(Lm0)*diag_Mm*Lm0_partial(1:end,1:end,i);
    M0_partial(1:b,1:b,i)= iota0'*(temp1+temp2)*iota0; %6x6 %equation 117 of TRO
end
